simulink model "m7_reactor_alara_closed_loop"  (R2026b)
settings: Solver=ode45  StopTime=25.0
settings Model: Creator=aurascoper  LastModifiedBy=aurascoper

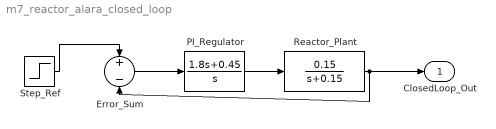
== system m7_reactor_alara_closed_loop ==
  Error_Sum : Sum  Inputs=+-
  PI_Regulator : TransferFcn  Numerator=[1.8 0.45]  Denominator=[1.0 0.0]
  Reactor_Plant : TransferFcn  Numerator=[0.15]  Denominator=[1.0 0.15]
  Step_Ref : Step  Time=0  SampleTime=0
  ClosedLoop_Out : Outport
  wires:
  Step_Ref/1 -> Error_Sum/1
  Error_Sum/1 -> PI_Regulator/1
  PI_Regulator/1 -> Reactor_Plant/1
  Reactor_Plant/1 -> ClosedLoop_Out/1, Error_Sum/2
